simulink model "lab9_simulink"  (R2021b)
settings: Solver=VariableStepAuto  StartTime=0.0  StopTime=24.0  RelTol=1e-3
settings Model: Creator=13676840  LastModifiedBy=13676840

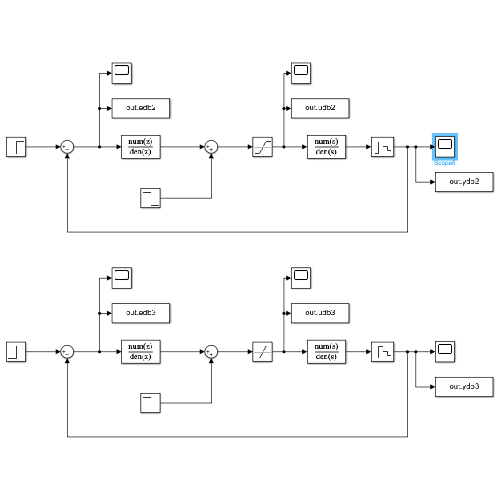
[thumbnail: Simulink's stored preview of the top-level diagram]
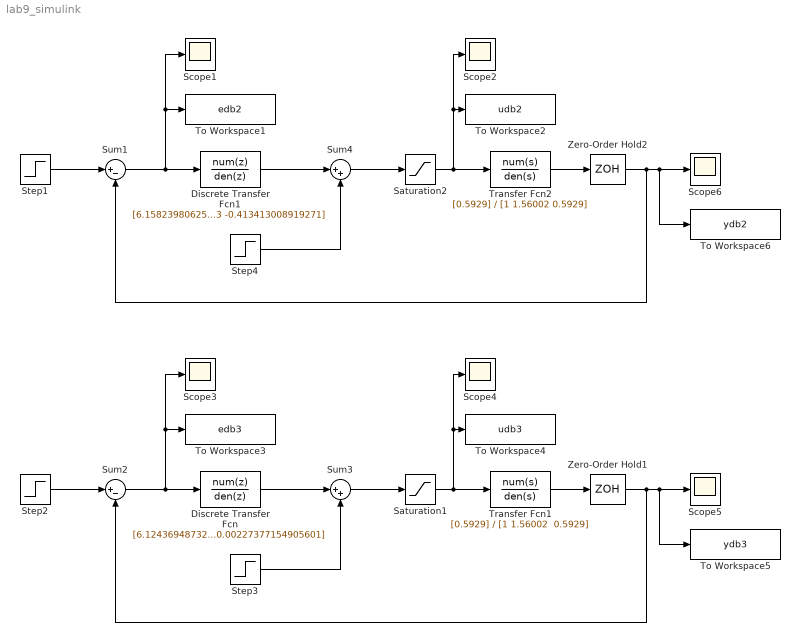
== system lab9_simulink ==
  Discrete Transfer Fcn : DiscreteTransferFcn  Numerator=[6.12436948732201 -7.24171746016698 2.10548125529365 -0.0402370364857296]  Denominator=[1 -0.583360762629786 -0.414365465821159 -0.00227377154905601]  SampleTime=0.6723
  Discrete Transfer Fcn1 : DiscreteTransferFcn  Numerator=[6.15823980625643 -7.31582481558712 2.1575850093307]  Denominator=[1 -0.58658699108073 -0.413413008919271]  SampleTime=0.6723
  Saturation1 : Saturate  UpperLimit=10  LowerLimit=-10
  Saturation2 : Saturate  UpperLimit=10  LowerLimit=-10
  Scope{1..6} (6 alike) : Scope
  Step1 : Step  Time=0  After=1.17  SampleTime=0
  Step2 : Step  Time=0  After=1.17  SampleTime=0
  Step3 : Step  Time=12  After=-0.15  SampleTime=0
  Step4 : Step  Time=12  After=-0.15  SampleTime=0
  Sum1 : Sum  Inputs=|+-
  Sum2 : Sum  Inputs=|+-
  Sum3 : Sum  Inputs=|++
  Sum4 : Sum  Inputs=|++
  To Workspace1 : ToWorkspace  VariableName=edb2  SaveFormat=Timeseries  SampleTime=-1
  To Workspace2 : ToWorkspace  VariableName=udb2  SaveFormat=Timeseries  SampleTime=-1
  To Workspace3 : ToWorkspace  VariableName=edb3  SaveFormat=Timeseries  SampleTime=-1
  To Workspace4 : ToWorkspace  VariableName=udb3  SaveFormat=Timeseries  SampleTime=-1
  To Workspace5 : ToWorkspace  VariableName=ydb3  SaveFormat=Timeseries  SampleTime=-1
  To Workspace6 : ToWorkspace  VariableName=ydb2  SaveFormat=Timeseries  SampleTime=-1
  Transfer Fcn1 : TransferFcn  Numerator=[0.5929]  Denominator="[1 1.56002  0.5929]"
  Transfer Fcn2 : TransferFcn  Numerator=[0.5929]  Denominator=[1 1.56002 0.5929]
  Zero-Order Hold1 : ZeroOrderHold  SampleTime=0.6723
  Zero-Order Hold2 : ZeroOrderHold  SampleTime=0.6723
  wires:
  Transfer Fcn1/1 -> Zero-Order Hold1/1
  Saturation1/1 -> To Workspace4/1, Scope4/1, Transfer Fcn1/1
  Sum2/1 -> Discrete Transfer Fcn/1, To Workspace3/1, Scope3/1
  Zero-Order Hold1/1 -> Sum2/2, To Workspace5/1, Scope5/1
  Sum3/1 -> Saturation1/1
  Step2/1 -> Sum2/1
  Step3/1 -> Sum3/2
  Discrete Transfer Fcn/1 -> Sum3/1
  Step4/1 -> Sum4/2
  Step1/1 -> Sum1/1
  Sum4/1 -> Saturation2/1
  Discrete Transfer Fcn1/1 -> Sum4/1
  Zero-Order Hold2/1 -> Sum1/2, To Workspace6/1, Scope6/1
  Sum1/1 -> Discrete Transfer Fcn1/1, To Workspace1/1, Scope1/1
  Saturation2/1 -> To Workspace2/1, Scope2/1, Transfer Fcn2/1
  Transfer Fcn2/1 -> Zero-Order Hold2/1
